simulink model "source_test"  (R2023b)
settings: Solver=FixedStepDiscrete  StartTime=0.0  StopTime=(N-1)*Tb  FixedStep=Tb  RelTol=1e-3
values from neighbouring files (symbols this model uses):
  graine = P.graine    [parametres.m]    (also in parametres_perso.m = mod(sum(c .* (1:numel(c)) * 31) + 7 * numel(c), 2^31 - 1); partie2_1.m)
  p1 = P.p1    [parametres.m]    (also in partie2_1.m; partie2_4_q9.m = mean(bits))
  Tb = 1    [parametres.m]    (also in partie2_1.m)
libraries: simulink x1
settings Model: Creator=e2507477  LastModifiedBy=e2507477

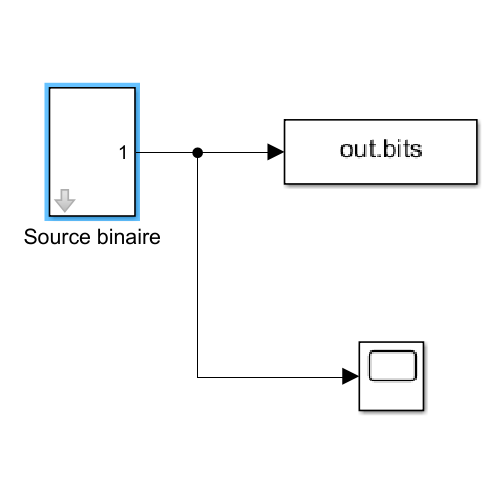
[thumbnail: Simulink's stored preview of the top-level diagram]
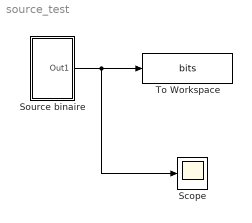
== system source_test ==
  Scope : Scope
  Source binaire : Subsystem  mask{p1=p1, Tb=Tb, graine=graine}
      mask prompts: p1 "probabilite d'emetre un 1"; Tb "duree d'un bit Tb"
  To Workspace : ToWorkspace  VariableName=bits  SampleTime=-1
  wires:
  Source binaire/1(Out1) -> Scope/1, To Workspace/1

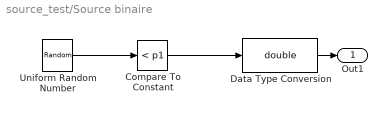
== system source_test/Source binaire ==
  Compare To Constant : simulink/Logic and Bit Operations/Compare To Constant  relop=<  const=p1  OutDataTypeStr=boolean
  Data Type Conversion : DataTypeConversion  OutDataTypeStr=double  SaturateOnIntegerOverflow=off  RndMeth=Floor
  Uniform Random Number : UniformRandomNumber  Minimum=0  Seed=graine  SampleTime=Tb
  Out1 : Outport
  wires:
  Uniform Random Number/1 -> Compare To Constant/1
  Compare To Constant/1 -> Data Type Conversion/1
  Data Type Conversion/1 -> Out1/1
